simulink model "LCC_Controller"  (R2026b)
settings: Solver=FixedStepDiscrete  StopTime=inf  FixedStep=0.02
InitFcn:
  | lcc_controller_init;
values from neighbouring files (symbols this model uses):
  C = lcc_controller_params()    [build_lcc_controller.m]    (also in identify_lcc_plant.m = struct([]); lcc_controller_init.m)
libraries: mpclib x1
settings Model: Creator=kikiw  LastModifiedBy=kikiw
settings OptimizationCC: DefaultParameterBehavior=Inlined  DifferentSizesBufferReuse=on  EfficientTunableParamExpr=on  EnhancedBackFolding=on  OptimizationCustomize=off  OptimizeBlockOrder=speed  PassReuseOutputArgsAs=Individual arguments  RemoveInternalMemoryZeroInit=on  RemoveRootLevelIOMemoryZeroInit=on
settings DebuggingCC: ParameterTunabilityLossMsg=error
settings SFSimCC: MATLABDynamicMemAlloc=off
settings RTWCC: DataTypeReplacement=CDataTypesFixedWidth  Description=Embedded Coder  GenerateReport=on  SystemTargetFile=ert.tlc  TargetLang=C++  TemplateMakefile=ert_default_tmf
settings CodeAppCC: ForceParamTrailComments=on  IgnoreCustomStorageClasses=off  InsertBlockDesc=on  OperatorAnnotations=on  SFDataObjDesc=on  SimulinkDataObjDesc=on
settings ERTTargetCC: CodeInterfacePackaging=C++ class  CombineSignalStateStructs=on  GenerateSampleERTMain=on  MaxIdInt16=INT16_MAX  MaxIdInt32=INT32_MAX  MaxIdInt64=INT64_MAX  MaxIdInt8=INT8_MAX  MaxIdUint16=UINT16_MAX  MaxIdUint32=UINT32_MAX  MaxIdUint64=UINT64_MAX  MaxIdUint8=UINT8_MAX  MinIdInt16=INT16_MIN  MinIdInt32=INT32_MIN  MinIdInt64=INT64_MIN  MinIdInt8=INT8_MIN  RootIOFormat=Structure reference  SubcomponentCodeInterfacePackaging=C++ class  TargetLangStandard=C++11 (ISO)
settings CPPComponent: ExternalIOMemberVisibility=private  GenerateDestructor=on  GenerateExternalIOAccessMethods=Inlined structure-based method  GenerateInternalMemberAccessMethods=None  GenerateParameterAccessMethods=None  IncludeModelTypesInModelClass=on  InternalMemberVisibility=private  ParameterMemberVisibility=private  UseOperatorNewForModelRefRegistration=off

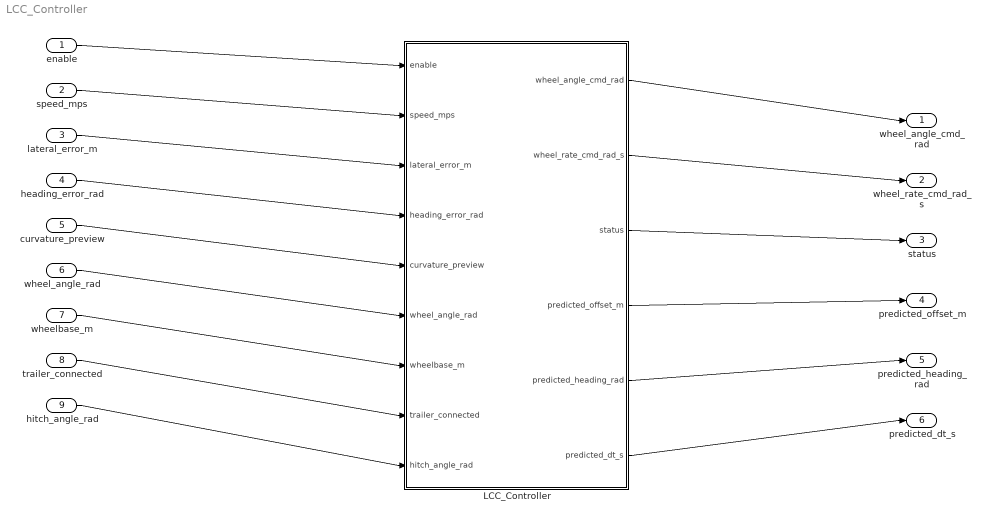
== system LCC_Controller ==
  enable : Inport  OutDataTypeStr=boolean  PortDimensions=1  SampleTime=C.Ts
  speed_mps : Inport  Port=2  OutDataTypeStr=double  PortDimensions=1  SampleTime=C.Ts
  lateral_error_m : Inport  Port=3  OutDataTypeStr=double  PortDimensions=1  SampleTime=C.Ts
  heading_error_rad : Inport  Port=4  OutDataTypeStr=double  PortDimensions=1  SampleTime=C.Ts
  curvature_preview : Inport  Port=5  OutDataTypeStr=double  PortDimensions=61  SampleTime=C.Ts
  wheel_angle_rad : Inport  Port=6  OutDataTypeStr=double  PortDimensions=1  SampleTime=C.Ts
  wheelbase_m : Inport  Port=7  OutDataTypeStr=double  PortDimensions=1  SampleTime=C.Ts
  trailer_connected : Inport  Port=8  OutDataTypeStr=boolean  PortDimensions=1  SampleTime=C.Ts
  hitch_angle_rad : Inport  Port=9  OutDataTypeStr=double  PortDimensions=1  SampleTime=C.Ts
  LCC_Controller : Subsystem  TreatAsAtomicUnit=on
  wheel_angle_cmd_rad : Outport  OutDataTypeStr=double  PortDimensions=1
  wheel_rate_cmd_rad_s : Outport  Port=2  OutDataTypeStr=double  PortDimensions=1
  status : Outport  Port=3  OutDataTypeStr=uint8  PortDimensions=1
  predicted_offset_m : Outport  Port=4  OutDataTypeStr=double  PortDimensions=16
  predicted_heading_rad : Outport  Port=5  OutDataTypeStr=double  PortDimensions=16
  predicted_dt_s : Outport  Port=6  OutDataTypeStr=double  PortDimensions=1
  wires:
  enable/1 -> LCC_Controller/1(enable)
  speed_mps/1 -> LCC_Controller/2(speed_mps)
  lateral_error_m/1 -> LCC_Controller/3(lateral_error_m)
  heading_error_rad/1 -> LCC_Controller/4(heading_error_rad)
  curvature_preview/1 -> LCC_Controller/5(curvature_preview)
  wheel_angle_rad/1 -> LCC_Controller/6(wheel_angle_rad)
  wheelbase_m/1 -> LCC_Controller/7(wheelbase_m)
  trailer_connected/1 -> LCC_Controller/8(trailer_connected)
  hitch_angle_rad/1 -> LCC_Controller/9(hitch_angle_rad)
  LCC_Controller/1(wheel_angle_cmd_rad) -> wheel_angle_cmd_rad/1
  LCC_Controller/2(wheel_rate_cmd_rad_s) -> wheel_rate_cmd_rad_s/1
  LCC_Controller/3(status) -> status/1
  LCC_Controller/4(predicted_offset_m) -> predicted_offset_m/1
  LCC_Controller/5(predicted_heading_rad) -> predicted_heading_rad/1
  LCC_Controller/6(predicted_dt_s) -> predicted_dt_s/1

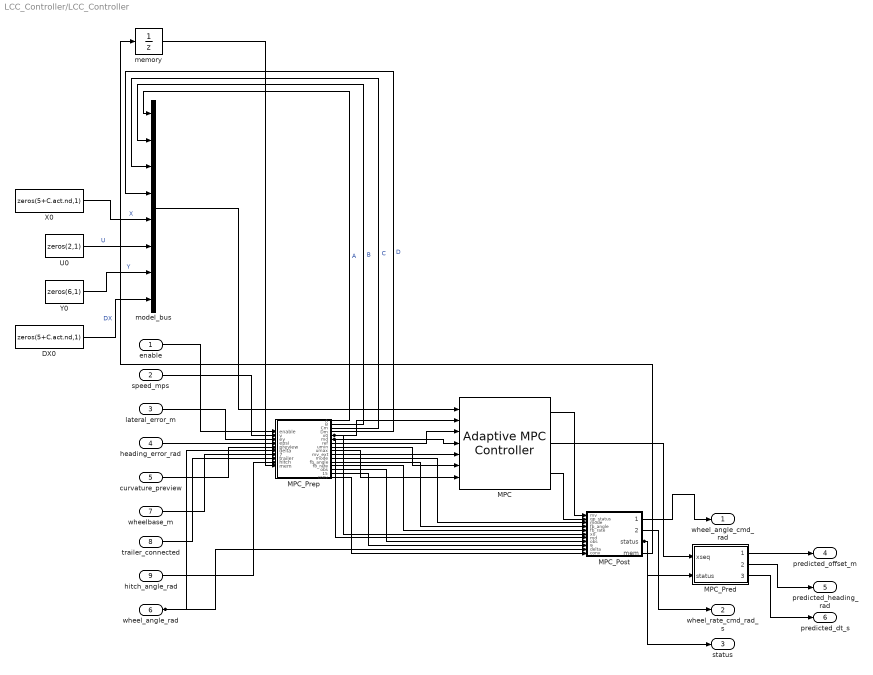
== system LCC_Controller/LCC_Controller ==
  enable : Inport
  speed_mps : Inport  Port=2
  lateral_error_m : Inport  Port=3
  heading_error_rad : Inport  Port=4
  curvature_preview : Inport  Port=5
  wheel_angle_rad : Inport  Port=6
  wheelbase_m : Inport  Port=7
  trailer_connected : Inport  Port=8
  hitch_angle_rad : Inport  Port=9
  DX0 : Constant  Value=zeros(5+C.act.nd,1)  VectorParams1D=off  SampleTime=C.Ts
  MPC : mpclib/Adaptive MPC Controller  SCDEnableBlockLinearizationSpecification=on  mpcobj=mpcLcc  enable_value=0  updateMPCinCallerWorkspace=on  md_inport=on  mv_inport=on  uref_inport=off  return_cost=off  return_mvseq=off  return_qpstatus=on  return_xseq=on  return_state=off  return_ovseq=off  state_inport=on  isltv_plant=off  umin_inport=on  umax_inport=on  ymin_inport=off  ymax_inport=off  cc_inport=off  ywt_inport=off  uwt_inport=off  duwt_inport=off  rhoeps_inport=off  pm_inport=off  MaximumP=10  HorizonChoice=FixedHorizon  BlockDataType=double  SampleTimeInherited=off  switch_inport=off
  MPC_Post : MATLAB Function  TreatAsAtomicUnit=on
  MPC_Pred : MATLAB Function  TreatAsAtomicUnit=on
  MPC_Prep : MATLAB Function  TreatAsAtomicUnit=on
  U0 : Constant  Value=zeros(2,1)  VectorParams1D=off  SampleTime=C.Ts
  X0 : Constant  Value=zeros(5+C.act.nd,1)  VectorParams1D=off  SampleTime=C.Ts
  Y0 : Constant  Value=zeros(6,1)  VectorParams1D=off  SampleTime=C.Ts
  memory : UnitDelay  InitialCondition=zeros(C.mem_n,1)  SampleTime=C.Ts
  model_bus : BusCreator  Inputs=8
  wheel_angle_cmd_rad : Outport
  wheel_rate_cmd_rad_s : Outport  Port=2
  status : Outport  Port=3
  predicted_offset_m : Outport  Port=4
  predicted_heading_rad : Outport  Port=5
  predicted_dt_s : Outport  Port=6
  wires:
  enable/1 -> MPC_Prep/1(enable)
  speed_mps/1 -> MPC_Prep/2(v)
  DX0/1 -> model_bus/8  "DX"
  model_bus/1 -> MPC/1
  Y0/1 -> model_bus/7  "Y"
  U0/1 -> model_bus/6  "U"
  MPC_Post/2(wheel_rate_cmd) -> wheel_rate_cmd_rad_s/1
  X0/1 -> model_bus/5  "X"
  wheel_angle_rad/1 -> MPC_Post/10(delta), MPC_Prep/6(delta)
  curvature_preview/1 -> MPC_Prep/5(preview)
  heading_error_rad/1 -> MPC_Prep/4(epsi)
  lateral_error_m/1 -> MPC_Prep/3(ey)
  memory/1 -> MPC_Prep/10(mem)
  MPC_Pred/3(pred_dt) -> predicted_dt_s/1
  hitch_angle_rad/1 -> MPC_Prep/9(hitch)
  trailer_connected/1 -> MPC_Prep/8(trailer)
  wheelbase_m/1 -> MPC_Prep/7(wheelbase)
  MPC_Prep/1(A) -> model_bus/1  "A"
  MPC_Prep/2(B) -> model_bus/2  "B"
  MPC_Prep/3(Cm) -> model_bus/3  "C"
  MPC_Prep/4(Dm) -> model_bus/4  "D"
  MPC_Prep/5(x0) -> MPC_Post/6(x0), MPC/2
  MPC_Prep/6(md) -> MPC_Post/7(md), MPC/4
  MPC_Prep/7(ref) -> MPC/3
  MPC_Prep/8(umin) -> MPC/6
  MPC_Prep/9(umax) -> MPC/7
  MPC_Pred/1(pred_ey) -> predicted_offset_m/1
  MPC_Prep/10(mv_ext) -> MPC/5
  MPC_Prep/11(mode) -> MPC_Post/3(mode)
  MPC_Prep/12(fb_angle) -> MPC_Post/4(fb_angle)
  MPC_Prep/13(fb_rate) -> MPC_Post/5(fb_rate)
  MPC_Prep/14(obs) -> MPC_Post/8(obs)
  MPC_Prep/15(pred_rows) -> MPC_Post/9(pred_rows)
  MPC_Prep/16(conv) -> MPC_Post/11(conv)
  MPC/1 -> MPC_Post/1(mv)
  MPC/2 -> MPC_Pred/1(xseq)
  MPC_Pred/2(pred_epsi) -> predicted_heading_rad/1
  MPC/3 -> MPC_Post/2(qp_status)
  MPC_Post/1(wheel_angle_cmd) -> wheel_angle_cmd_rad/1
  MPC_Post/3(status) -> MPC_Pred/2(status), status/1
  MPC_Post/4(mem) -> memory/1

== matlab function LCC_Controller/MPC_Post ==
  data: mv input; wheel_angle_cmd output; qp_status input; mode input; fb_angle input; fb_rate input; x0 input; md input; obs input; pred_rows input; delta input; conv input; wheel_rate_cmd output; status output; mem output; C parameter
function [wheel_angle_cmd, wheel_rate_cmd, status, mem] = MPC_Post(mv, qp_status, mode, fb_angle, fb_rate, x0, md, obs, pred_rows, delta, conv, C)
[wheel_angle_cmd, wheel_rate_cmd, status, mem] = lcc_mpc_post(mv, qp_status, mode, fb_angle, fb_rate, x0, md(1), obs, pred_rows, delta, conv, C);

== matlab function LCC_Controller/MPC_Prep ==
  data: enable input; A output; v input; ey input; epsi input; preview input; delta input; wheelbase input; trailer input; hitch input; mem input; B output; Cm output; Dm output; x0 output; md output; ref output; umin output; umax output; mv_ext output; mode output; fb_angle output; fb_rate output; obs output; pred_rows output; conv output; C parameter
function [A, B, Cm, Dm, x0, md, ref, umin, umax, mv_ext, mode, fb_angle, fb_rate, obs, pred_rows, conv] = MPC_Prep(enable, v, ey, epsi, preview, delta, wheelbase, trailer, hitch, mem, C)
[A, B, Cm, Dm, x0, md, ref, umin, umax, mv_ext, mode, fb_angle, fb_rate, obs, pred_rows, conv] = lcc_mpc_prep(enable, v, ey, epsi, preview, delta, wheelbase, trailer, hitch, mem, C);

== matlab function LCC_Controller/MPC_Pred ==
  data: xseq input; pred_ey output; status input; pred_epsi output; pred_dt output; C parameter
function [pred_ey, pred_epsi, pred_dt] = MPC_Pred(xseq, status, C)
[pred_ey, pred_epsi, pred_dt] = lcc_mpc_pred(xseq, status, C);
